simulink model "KUKA_coupled"  (R2021b)
settings: Solver=ode4  StartTime=0.0  StopTime=0.01  FixedStep=0.01  RelTol=1e-3  EnableMultiTasking=on
InitFcn:
  | % ************** Initiate forces
  | % f0=[0;0;0;0;0;0];
  | % f0=[0;0;0;0;0;0;0];
  | %f_0=[0;0;0];
  | %f_m=[0;0];
  | %f_e=[0;0;0;0;0;0];
  | %iota0=eye(6);
  | % ************** Initiate states
  | %q_m=[2;1];
  | %q_dot_m=[0;1];
  | %P=[0;0;0];
  | %V_I0=[0;0;0];
  | % ************** Load main
  | %run(Main.m)
StopFcn:
  | %format long
  | %table(out.qddot.data(:,1)',out.qddot_ref.data(1,:))
values from neighbouring files (symbols this model uses):
  diag_M = diagonalize(M_frak0, M_frak)    [Create_Robot.m]    (also in Main.m; Main__iiwa7.m; diagonalize.m = zeros(6*(n+1),6*(n+1)); test_C_Main.m)
  f_0 = [0;0;0]    [Create_Robot.m]    (also in Main.m; Main__iiwa7.m = [0;0;0;0;0;0]; test_C_Main.m)
  f_e = [0;0;0;0;0;0]    [Create_Robot.m]    (also in Main.m = [0;0;0]; Main__iiwa7.m; test_C_Main.m)
  f_m = [0;0]    [Create_Robot.m]    (also in Main.m; Main__iiwa7.m; test_C_Main.m)
  I0 = eye(3)*416.667    [Create_Robot.m]    (also in Main.m; Main__iiwa7.m = eye(3)*1.66667; test_C_Main.m)
  iota0 = [1 0 0; 0 1 0;zeros(3,3);0 0 1]    [Create_Robot.m]    (also in Main.m = [1 0 0 0 0 0; 0 1 0 0 0 0; 0 0 0 0 0 1]'; Main__iiwa7.m = eye(6,6); test_C_Main.m)
  m0 = 100    [Create_Robot.m]    (also in Main.m; Main__iiwa7.m = 10; test_C_Main.m)
  P = [0;0;0]    [Create_Robot.m]    (also in Main.m = M0*V_I0+M0m*q_dot_m; Main__iiwa7.m = M0*V_I0+M0m*q_dot_m; test_C_Main.m)
  q_dot_m = [0;0]    [Create_Robot.m]    (also in Main.m; Main__iiwa7.m; test_C_Main.m)
  q_m = [0;0]    [Create_Robot.m]    (also in Main.m = [0.2;0.4]; Main__iiwa7.m = [0.2;0.4]; test_C_Main.m = [1;0])
  sc_size = 5    [Main.m]    (also in Main__iiwa7.m = 1)
  X = [0 -x(3) x(2) ; x(3) 0 -x(1) ; -x(2) x(1) 0 ]    [skewsym.m]
  Xi_m_matrix = zeros(6*n,n)    [Create_Robot.m]    (also in Main.m; Main__iiwa7.m; test_C_Main.m)
undefined symbols (not defined in the file or in its folder): rho_0t, V_0t, Xi_m, Y, Z
libraries: sm_lib x87, nesl_utility x51, robotcorelib x2
(part 1 of 3)
settings Model: Creator=Bmmog  LastModifiedBy=Bmmog
settings SimscapeCC: SimscapeLogType=all
settings ExplorerConfigSet: InternalSimMechanicsExplorerSettings="<ExplorerConfiguration><canonicalview>default</canonicalview><AnimationSetting><BasePlaybackSpeed>1.0</BasePlaybackSpeed><PlaybackSpeedFactor>1.0</PlaybackSpeedFactor></AnimationSetting><TilePanel><TileInfo><Tiles Columns=\"1\" Count=\"1\" Rows=\"1\"><Column Weight=\"1\"/><Row Weight=\"1\"/><Tile Height=\"1\" Width=\"1\" X=\"0\" Y=\"0\"/></Tiles></TileInfo><SceneInfo><SceneViewer><BGColor><R>1</R><G>1</G><B>1</B></BGColor><Camera><DoPerspective>off</DoPerspective><Position><X>-2.86799693255843557</X><Y>0.354289043707541051</Y><Z>3.4484382025260043</Z></Position><Center><X>-0.226627357164881998</X><Y>-0.0947422938384068769</Y><Z>1.20474693109606124</Z></Center><Up><X>0.463975295415888944</X><Y>0.796982789726579544</Y><Z>0.386710949060636133</Z></Up><ViewLimDist>1</ViewLimDist><YLim>1.02199972307052578</YLim><XLim>1.06112681813448173</XLim></Camera></SceneViewer></SceneInfo></TilePanel><MechEditorPanel><Cameras/><GfxPanelCameraMap/><VideoCreator><PlaybackSpeedRatio>1.0</PlaybackSpeedRatio><FrameRate>30</FrameRate><VideoFormat>Motion JPEG AVI</VideoFormat><FrameSize>auto</FrameSize></VideoCreator></MechEditorPanel></ExplorerConfiguration>"

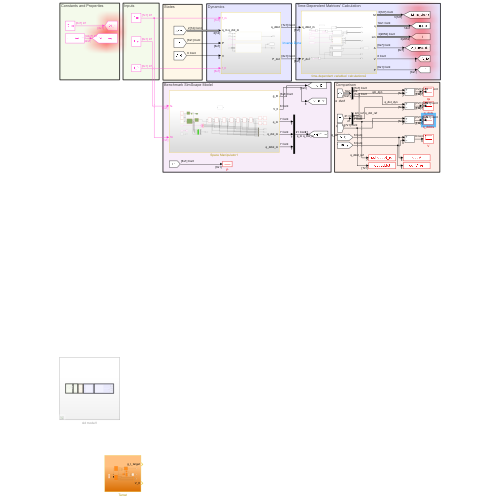
[thumbnail: Simulink's stored preview of the top-level diagram]
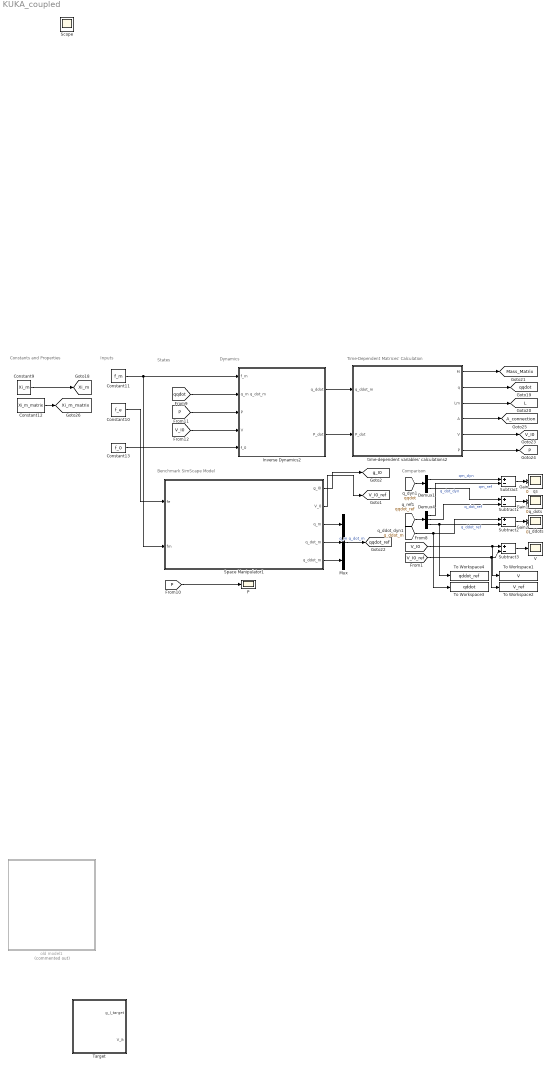
== system KUKA_coupled ==
  note: Benchmark SimScape Model
  note: Time-Dependent Matrices' Calculation
  note: Comparison
  note: States
  note: Constants and Properties
  note: Inputs
  note: Dynamics
  Constant10 : Constant  Value=f_e  VectorParams1D=off
  Constant11 : Constant  Value=f_m  VectorParams1D=off
  Constant12 : Constant  Value=Xi_m_matrix  VectorParams1D=off
  Constant13 : Constant  Value=f_0  VectorParams1D=off
  Constant9 : Constant  Value=Xi_m  VectorParams1D=off
  Demux1 : Demux  Outputs=2
  Demux4 : Demux  Outputs=3
  Gain : Gain  Gain=0
  Gain1 : Gain  Gain=0
  Gain2 : Gain  Gain=0
  Inverse Dynamics2 : Subsystem
  Mux : Mux  Inputs=3
  P : Scope
  Space Manipulator1 : Subsystem
  Subtract{,1..3} (4 alike) : Sum  Inputs=+-
  Target : Subsystem
  To Workspace1 : ToWorkspace  VariableName=V  SaveFormat=Timeseries  SampleTime=-1
  To Workspace2 : ToWorkspace  VariableName=V_ref  SaveFormat=Timeseries  SampleTime=-1
  To Workspace3 : ToWorkspace  VariableName=qddot  SaveFormat=Timeseries  SampleTime=-1
  To Workspace4 : ToWorkspace  VariableName=qddot_ref  SaveFormat=Timeseries  SampleTime=-1
  V : Scope
  old model1 : Subsystem  Commented=on
  q_ddots : Scope
  q_dots : Scope
  qs : Scope
  time-dependent variables' calculations2 : Subsystem
  Scope : Scope
  tag scope: A_connection=global, L=global, Mass_Matrix=global, P=global, V_I0=global, V_I0_ref=global, Xi_m=global, Xi_m_matrix=global, g_I0=global, qqdot=global, qqdot_ref=global
  wires:
  [P] -> P/1
  Constant10/1 -> Space Manipulator1/1(fe)
  Constant12/1 -> [Xi_m_matrix]
  [qqdot] -> Demux1/1
  Inverse Dynamics2/1(q_ddot) -> time-dependent variables' calculations2/1(q_ddot_m)
  Demux1/1 -> Subtract/1  "qm_dyn"
  Demux4/1 -> Subtract/2  "qm_ref"
  [qqdot_ref] -> Demux4/1
  Space Manipulator1/4(q_dot_m) -> Mux/2
  time-dependent variables' calculations2/1(M) -> [Mass_Matrix]
  Constant9/1 -> [Xi_m]
  Constant11/1 -> Space Manipulator1/2(fm), Inverse Dynamics2/1(f_m)
  [q_ddot_m] -> Subtract2/1, To Workspace3/1
  [qqdot] -> Inverse Dynamics2/2(q_m q_dot_m)
  Mux/1 -> [qqdot_ref]  "q_m q_dot_m"
  Demux1/2 -> Subtract1/1  "q_dot_dyn"
  Space Manipulator1/3(q_m) -> Mux/1
  [V_I0] -> Inverse Dynamics2/4(V)
  [V_I0] -> To Workspace1/1, Subtract3/1
  Inverse Dynamics2/2(P_dot) -> time-dependent variables' calculations2/2(P_dot)
  time-dependent variables' calculations2/6(P) -> [P]
  time-dependent variables' calculations2/3(Lm) -> [L]
  [P] -> Inverse Dynamics2/3(P)
  time-dependent variables' calculations2/5(V) -> [V_I0]
  Constant13/1 -> Inverse Dynamics2/5(f_0)
  time-dependent variables' calculations2/4(A) -> [A_connection]
  Demux4/3 -> Subtract2/2, To Workspace4/1  "q_ddot_ref"
  time-dependent variables' calculations2/2(q) -> [qqdot]
  Space Manipulator1/5(q_ddot_m) -> Mux/3
  Demux4/2 -> Subtract1/2  "q_dot_ref"
  Space Manipulator1/2(V_0) -> [V_I0_ref]
  [V_I0_ref] -> To Workspace2/1, Subtract3/2
  Subtract/1 -> Gain/1
  Subtract1/1 -> Gain1/1
  Subtract2/1 -> Gain2/1
  Subtract3/1 -> V/1
  Space Manipulator1/1(g_I0) -> [g_I0]
  Gain/1 -> qs/1
  Gain1/1 -> q_dots/1
  Gain2/1 -> q_ddots/1

== system KUKA_coupled/Inverse Dynamics2 ==
  f_m : Inport
  q_m q_dot_m : Inport  Port=2
  P : Inport  Port=3
  V : Inport  Port=4
  f_0 : Inport  Port=5
  Euler Poincare : Subsystem
  Internal Dynamics : Subsystem
  q_ddot : Outport
  P_dot : Outport  Port=2
  tag scope: q_ddot_m=global
  wires:
  f_m/1 -> Internal Dynamics/1(f_m)
  q_m q_dot_m/1 -> Internal Dynamics/2(q_m q_dot_m)
  Internal Dynamics/1(q_ddot) -> [q_ddot_m], q_ddot/1  "q_ddot"
  Euler Poincare/1(P_dot) -> P_dot/1  "P_dot"
  f_0/1 -> Euler Poincare/3(f_0)
  P/1 -> Internal Dynamics/3(P), Euler Poincare/1(P)
  V/1 -> Euler Poincare/2(V)

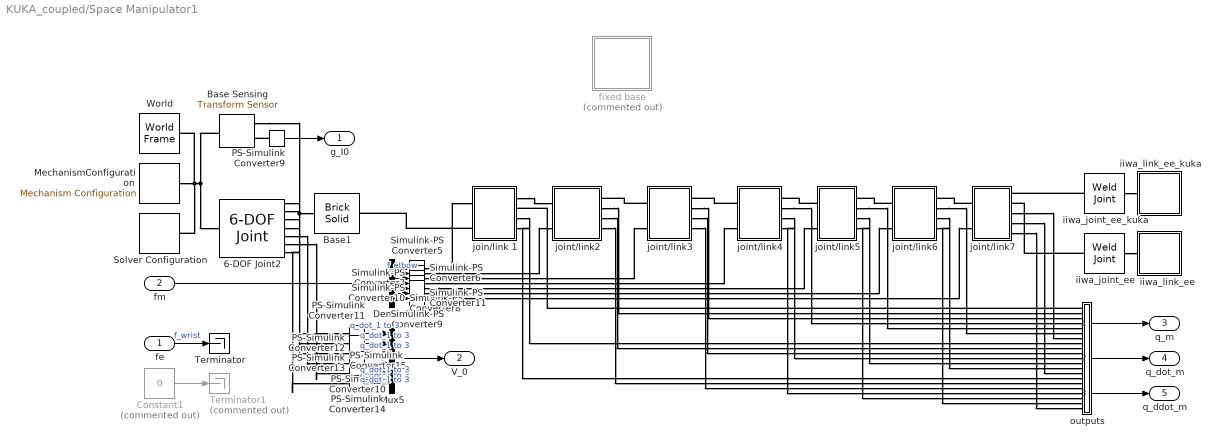
== system KUKA_coupled/Space Manipulator1 ==
  fe : Inport
  fm : Inport  Port=2
  6-DOF Joint2 : sm_lib/Joints/6-DOF Joint  JointMode=Normal  SenseConstraintForce=off  SenseConstraintForceX=off  SenseConstraintForceY=off  SenseConstraintForceZ=off  SenseConstraintTorque=off  SenseConstraintTorqueX=off  SenseConstraintTorqueY=off  SenseConstraintTorqueZ=off  SenseTotalForce=off  SenseTotalForceX=off  SenseTotalForceY=off  SenseTotalForceZ=off  SenseTotalTorque=off  SenseTotalTorqueX=off  SenseTotalTorqueY=off  SenseTotalTorqueZ=off  CompositeWrenchDir=FollowerOnBase  CompositeWrenchFrame=BaseFrame  PxEquilibriumPosition=0  PxEquilibriumPositionUnits=m  PxSpringStiffness=0  PxSpringStiffnessUnits=N/m  PxDampingCoefficient=0  PxDampingCoefficientUnits=N/(m/s)  PxTorqueActuationMode=NoTorque  PxMotionActuationMode=ComputedMotion  PxSensePosition=off  PxSenseVelocity=on  PxSenseAcceleration=off  PxSenseTorqueForce=off  PxSenseLowerLimitTorqueForce=off  PxSenseUpperLimitTorqueForce=off  PxLowerLimitSpecify=off  PxLowerLimitBound=-1  PxLowerLimitBoundUnits=m  PxLowerLimitStiffness=1e6  PxLowerLimitStiffnessUnits=N/m  PxLowerLimitDamping=1e3  PxLowerLimitDampingUnits=N/(m/s)  PxLowerLimitTransitionRegionWidth=1e-4  PxLowerLimitTransitionRegionWidthUnits=m  PxUpperLimitSpecify=off  PxUpperLimitBound=1  PxUpperLimitBoundUnits=m  PxUpperLimitStiffness=1e6  PxUpperLimitStiffnessUnits=N/m  PxUpperLimitDamping=1e3  PxUpperLimitDampingUnits=N/(m/s)  PxUpperLimitTransitionRegionWidth=1e-4  PxUpperLimitTransitionRegionWidthUnits=m  PxPositionTargetSpecify=on  PxPositionTargetPriority=High  PxPositionTargetValue=0  PxPositionTargetValueUnits=m  PxVelocityTargetSpecify=off  PxVelocityTargetPriority=High  PxVelocityTargetValue=0  PxVelocityTargetValueUnits=m/s  PyEquilibriumPosition=0  PyEquilibriumPositionUnits=m  PySpringStiffness=0  PySpringStiffnessUnits=N/m  PyDampingCoefficient=0  PyDampingCoefficientUnits=N/(m/s)  PyTorqueActuationMode=NoTorque  PyMotionActuationMode=ComputedMotion  PySensePosition=off  PySenseVelocity=on  PySenseAcceleration=off  PySenseTorqueForce=off  PySenseLowerLimitTorqueForce=off  PySenseUpperLimitTorqueForce=off  PyLowerLimitSpecify=off  PyLowerLimitBound=-1  PyLowerLimitBoundUnits=m  PyLowerLimitStiffness=1e6  PyLowerLimitStiffnessUnits=N/m  PyLowerLimitDamping=1e3  PyLowerLimitDampingUnits=N/(m/s)  PyLowerLimitTransitionRegionWidth=1e-4  PyLowerLimitTransitionRegionWidthUnits=m  PyUpperLimitSpecify=off  PyUpperLimitBound=1  PyUpperLimitBoundUnits=m  PyUpperLimitStiffness=1e6  PyUpperLimitStiffnessUnits=N/m  PyUpperLimitDamping=1e3  PyUpperLimitDampingUnits=N/(m/s)  PyUpperLimitTransitionRegionWidth=1e-4  PyUpperLimitTransitionRegionWidthUnits=m  PyPositionTargetSpecify=on  PyPositionTargetPriority=High  PyPositionTargetValue=0  PyPositionTargetValueUnits=m  PyVelocityTargetSpecify=off  PyVelocityTargetPriority=High  PyVelocityTargetValue=0  PyVelocityTargetValueUnits=m/s  PzEquilibriumPosition=0  PzEquilibriumPositionUnits=m  PzSpringStiffness=0  PzSpringStiffnessUnits=N/m  PzDampingCoefficient=0  PzDampingCoefficientUnits=N/(m/s)  PzTorqueActuationMode=NoTorque  PzMotionActuationMode=ComputedMotion  PzSensePosition=off  PzSenseVelocity=on  PzSenseAcceleration=off  PzSenseTorqueForce=off  PzSenseLowerLimitTorqueForce=off  PzSenseUpperLimitTorqueForce=off  PzLowerLimitSpecify=off  PzLowerLimitBound=-1  PzLowerLimitBoundUnits=m  PzLowerLimitStiffness=1e6  PzLowerLimitStiffnessUnits=N/m  PzLowerLimitDamping=1e3  PzLowerLimitDampingUnits=N/(m/s)  PzLowerLimitTransitionRegionWidth=1e-4  PzLowerLimitTransitionRegionWidthUnits=m  PzUpperLimitSpecify=off  PzUpperLimitBound=1  PzUpperLimitBoundUnits=m  PzUpperLimitStiffness=1e6  PzUpperLimitStiffnessUnits=N/m  PzUpperLimitDamping=1e3  PzUpperLimitDampingUnits=N/(m/s)  PzUpperLimitTransitionRegionWidth=1e-4  PzUpperLimitTransitionRegionWidthUnits=m  PzPositionTargetSpecify=on  PzPositionTargetPriority=High  PzPositionTargetValue=0  PzPositionTargetValueUnits=m  PzVelocityTargetSpecify=off  PzVelocityTargetPriority=High  PzVelocityTargetValue=0  PzVelocityTargetValueUnits=m/s  SphDefPosRotationMethod=None  SphDefPosRotationAngleUnits=deg  SphDefPosRotationStandardAxis=+Z  SphDefPosRotationAngle=0.0  SphDefPosRotationArbitraryAxis=[0 0 1]  SphDefPosFollAlignAxisA=+X  SphDefPosBaseAlignAxisA=+Y  SphDefPosFollAlignAxisB=+Y  SphDefPosBaseAlignAxisB=+Z  SphDefPosRotationSequenceAxes=FollowerAxes  SphDefPosRotationSequence=XYX  SphDefPosRotationSequenceAngles=[0 0 0]  SphDefPosRotationSequenceAnglesUnits=deg  SphDefPosRotationMatrix=[1 0 0; 0 1 0; 0 0 1]  SphEqPosRotationMethod=None  SphEqPosRotationAngleUnits=deg  SphEqPosRotationStandardAxis=+Z  SphEqPosRotationAngle=0.0  SphEqPosRotationArbitraryAxis=[0 0 1]  SphEqPosFollAlignAxisA=+X  SphEqPosBaseAlignAxisA=+Y  SphEqPosFollAlignAxisB=+Y  SphEqPosBaseAlignAxisB=+Z  SphEqPosRotationSequenceAxes=FollowerAxes  SphEqPosRotationSequence=XYX  SphEqPosRotationSequenceAngles=[0 0 0]  SphEqPosRotationSequenceAnglesUnits=deg  SphEqPosRotationMatrix=[1 0 0; 0 1 0; 0 0 1]  SphSpringStiffness=0  SphSpringStiffnessUnits=N*m/deg  SphDampingCoefficient=0  SphDampingCoefficientUnits=N*m/(deg/s)  SphActuateTorqueX=off  SphActuateTorqueY=off  SphActuateTorqueZ=off  SphActuateTorque=off  SphTorqueActuationMode=NoTorque  SphMotionActuationMode=ComputedMotion  SphActuationFrame=BaseFrame  SphSensePosition=off  SphSenseVelocityX=on  SphSenseVelocityY=on  SphSenseVelocityZ=on  SphSenseVelocity=off  SphSenseAccelerationX=off  SphSenseAccelerationY=off  SphSenseAccelerationZ=off  SphSenseAcceleration=off  SphSenseTorqueX=off  SphSenseTorqueY=off  SphSenseTorqueZ=off  SphSenseTorqueForce=off  SphSenseLowerLimitTorqueMag=off  SphSenseUpperLimitTorqueMag=off  SphSensingFrame=BaseFrame  SphLowerLimitSpecify=off  SphLowerLimitBound=15  SphLowerLimitBoundUnits=deg  SphLowerLimitStiffness=1e4  SphLowerLimitStiffnessUnits=N*m/deg  SphLowerLimitDamping=10  SphLowerLimitDampingUnits=N*m/(deg/s)  SphLowerLimitTransitionRegionWidth=0.1  SphLowerLimitTransitionRegionWidthUnits=deg  SphUpperLimitSpecify=off  SphUpperLimitBound=45  SphUpperLimitBoundUnits=deg  SphUpperLimitStiffness=1e4  SphUpperLimitStiffnessUnits=N*m/deg  SphUpperLimitDamping=10  SphUpperLimitDampingUnits=N*m/(deg/s)  SphUpperLimitTransitionRegionWidth=0.1  SphUpperLimitTransitionRegionWidthUnits=deg  SphPositionTargetRotationMethod=RotationSequence  SphPositionTargetRotationAngleUnits=deg  SphPositionTargetRotationStandardAxis=+Z  SphPositionTargetRotationAngle=0.0  SphPositionTargetRotationArbitraryAxis=[0 0 1]  SphPositionTargetFollAlignAxisA=+X  SphPositionTargetBaseAlignAxisA=+Y  SphPositionTargetFollAlignAxisB=+Y  SphPositionTargetBaseAlignAxisB=+Z  SphPositionTargetRotationSequenceAxes=FollowerAxes  SphPositionTargetRotationSequence=ZYX  SphPositionTargetRotationSequenceAngles=[0 0 0]  SphPositionTargetRotationSequenceAnglesUnits=deg  SphPositionTargetRotationMatrix=[1 0 0; 0 1 0; 0 0 1]  SphPositionTargetSpecify=off  SphPositionTargetPriority=High  SphVelocityTargetValue=[0 0.5 0.5]  SphVelocityTargetValueUnits=rad/s  SphVelocityTargetSpecify=off  SphVelocityTargetPriority=High  SphVelocityTargetInFollowerFrame=on
  Base Sensing : sm_lib/Frames and Transforms/Transform Sensor  MeasurementFrame=Base  SenseAngle=off  SenseAxis=off  SenseAngle1=off  SenseAngle2=off  SenseAngle3=off  SenseQ=off  SenseR=on  SenseOmegaX=off  SenseOmegaY=off  SenseOmegaZ=off  SenseOmega1=off  SenseOmega2=off  SenseOmega3=off  SenseQDot=off  SenseRDot=off  SenseAlphaX=off  SenseAlphaY=off  SenseAlphaZ=off  SenseAlpha1=off  SenseAlpha2=off  SenseAlpha3=off  SenseQDDot=off  SenseRDDot=off  SenseX=off  SenseY=off  SenseZ=off  SenseRad=off  SenseAzim=off  SenseDist=off  SenseInc=off  SenseXDot=off  SenseYDot=off  SenseZDot=off  SenseRadDot=off  SenseAzimDot=off  SenseDistDot=off  SenseIncDot=off  SenseXDDot=off  SenseYDDot=off  SenseZDDot=off  SenseRadDDot=off  SenseAzimDDot=off  SenseDistDDot=off  SenseIncDDot=off
  Base1 : sm_lib/Body Elements/Brick Solid  GraphicAmbientColor=[0.15 0.15 0.15 1.0]  BasedOnType=Mass  BrickDimensions=[sc_size,sc_size,sc_size]  BrickDimensionUnits=m  CenterOfMass=[0 0 0]  CenterOfMassUnits=m  GraphicDiffuseColor=[0.5 0.5 0.5]  Density=1000  DensityUnits=kg/m^3  DoExposeReferenceFrame=on  GraphicEmissiveColor=[0.0 0.0 0.0 1.0]  ExportEntireGeometry=off  SerializedFrames=<Frames><Frame><Id>Frame1</Id><Value><Name>F1</Name><Origin><Source>GeometricFeature</Source><FeatureName>+z surface</FeatureName></Origin><PrimaryAxis><DefinedDirection>+X</DefinedDirection><Source>ReferenceFrame</Source><SourceDirection>+X</SourceDirection><FeatureName></FeatureName></PrimaryAxis><SecondaryAxis><DefinedDirection>+Z</DefinedDirection><Source>ReferenceFrame</Source><SourceDirection>+Z</SourceDirection><FeatureName></FeatureName></SecondaryAxis></Value></Frame></Frames>  MarkerShape=Sphere  MarkerSize=10  GraphicType=FromGeometry  InertiaType=CalculateFromGeometry  Mass=m0  MassUnits=kg  MomentsOfInertia=[I0(1,1) I0(2,2) I0(3,3)]  MomentsOfInertiaUnits=kg*m^2  GraphicOpacity=1.0  ProductsOfInertia=[0 0 0]  ProductsOfInertiaUnits=kg*m^2  GraphicShininess=75  GraphicSpecularColor=[0.5 0.5 0.5 1.0]  GraphicVisPropType=SimpleVisualProperties
  Constant1 : Constant  Commented=on  Value=0
  Demux2 : Demux  Outputs=7
  MechanismConfiguration : sm_lib/Utilities/Mechanism Configuration  UniformGravity=Constant  GravityVector=[0 0 0]  GravityUnits=m/s^2  LinearizationDelta=0.001  JointModeTransitionNonlinearIterations=2
  Mux5 : Mux  Inputs=6
  PS-Simulink Converter{9..15} (7 alike) : nesl_utility/PS-Simulink Converter  PhysicalDomain=network_engine_domain  SubClassName=ps_output  LeftPortType=input  RightPortType=output  PseudoPeriodic=off  Frequencies=[]  Unit=inherit  AffineConversion=off
      settings: SourceProductBaseCode=PW,SS
  Simulink-PS Converter{5..11} (7 alike) : nesl_utility/Simulink-PS Converter  PhysicalDomain=network_engine_domain  SubClassName=ps_input  LeftPortType=input  RightPortType=output  PseudoPeriodic=off  Frequencies=[]  NoiseDistribution=none  NoiseParameters=[]  Unit=1  AffineConversion=off  FilteringAndDerivatives=provide  SimscapeFilterOrder=1  InputFilterTimeConstant=0.001  UdotUserProvided=0
      settings: SourceProductBaseCode=PW,SS
  Solver Configuration : nesl_utility/Solver Configuration  PhysicalDomain=network_engine_domain  SubClassName=solver  LeftPortType=input  RightPortType=generic  Tones=[]  Harmonics=[]  SimulateNoise=off  Profile=off  UseLocalSampling=off  EnableSwitchedLinearOptims=on  FrequencyDomain=off  UseCCode=off  RelTol=0.001  AbsTol=0.001  MinStep=1e-09  ToWorkspace=off  RevertToSquareIcSolve=off  NumHomotopyIterations=100  PhasorMode=off  PhasorModeNumHarmonics=1  DoDC=off  ResidualTolerance=1e-09  UseLocalSolver=off  LocalSolverChoice=NE_BACKWARD_EULER_ADVANCER  LocalSolverSampleTime=0.001  DoFixedCost=off  MaxNonlinIter=3  MaxModeIter=2  ComputeImpulses=off  ImpulseIterations=2  LinearAlgebra=auto  EquationFormulation=NE_TIME_EF  DelaysMemoryBudget=1024  AutomaticFiltering=on  FilteringTimeConstant=0.001  PartitionStorageMethod=AS_NEEDED  PartitionMemoryBudget=1024  PartitionMethod=ROBUST
      settings: SourceProductBaseCode=PW,SS
  Terminator : Terminator
  Terminator1 : Terminator  Commented=on
  World : sm_lib/Frames and Transforms/World Frame
  fixed base : Subsystem  Commented=on
  iiwa_joint_ee : sm_lib/Joints/Weld Joint  JointMode=Normal  SenseConstraintForce=off  SenseConstraintForceX=off  SenseConstraintForceY=off  SenseConstraintForceZ=off  SenseConstraintTorque=off  SenseConstraintTorqueX=off  SenseConstraintTorqueY=off  SenseConstraintTorqueZ=off  SenseTotalForce=off  SenseTotalForceX=off  SenseTotalForceY=off  SenseTotalForceZ=off  SenseTotalTorque=off  SenseTotalTorqueX=off  SenseTotalTorqueY=off  SenseTotalTorqueZ=off  CompositeWrenchDir=FollowerOnBase  CompositeWrenchFrame=BaseFrame
  iiwa_joint_ee_kuka : sm_lib/Joints/Weld Joint  JointMode=Normal  SenseConstraintForce=off  SenseConstraintForceX=off  SenseConstraintForceY=off  SenseConstraintForceZ=off  SenseConstraintTorque=off  SenseConstraintTorqueX=off  SenseConstraintTorqueY=off  SenseConstraintTorqueZ=off  SenseTotalForce=off  SenseTotalForceX=off  SenseTotalForceY=off  SenseTotalForceZ=off  SenseTotalTorque=off  SenseTotalTorqueX=off  SenseTotalTorqueY=off  SenseTotalTorqueZ=off  CompositeWrenchDir=FollowerOnBase  CompositeWrenchFrame=BaseFrame
  iiwa_link_ee : Subsystem
  iiwa_link_ee_kuka : Subsystem
  join/link 1 : Subsystem
  joint/link2 : Subsystem
  joint/link3 : Subsystem
  joint/link4 : Subsystem
  joint/link5 : Subsystem
  joint/link6 : Subsystem
  joint/link7 : Subsystem
  outputs : Subsystem
  g_I0 : Outport
  V_0 : Outport  Port=2
  q_m : Outport  Port=3
  q_dot_m : Outport  Port=4
  q_ddot_m : Outport  Port=5
  wires:
  fe/1 -> Terminator/1  "f_wrist"
  Constant1/1 -> Terminator1/1
  PS-Simulink Converter12/1 -> Mux5/2  "q_dot_1 to 3"
  PS-Simulink Converter15/1 -> Mux5/6  "q_dot_1 to 3"
  Mux5/1 -> V_0/1
  PS-Simulink Converter13/1 -> Mux5/4  "q_dot_1 to 3"
  PS-Simulink Converter9/1 -> g_I0/1
  PS-Simulink Converter11/1 -> Mux5/1  "q_dot_1 to 3"
  PS-Simulink Converter14/1 -> Mux5/5  "q_dot_1 to 3"
  PS-Simulink Converter10/1 -> Mux5/3  "q_dot_1 to 3"
  fm/1 -> Demux2/1
  Demux2/3 -> Simulink-PS Converter7/1
  Demux2/1 -> Simulink-PS Converter5/1
  Demux2/6 -> Simulink-PS Converter10/1
  Demux2/5 -> Simulink-PS Converter9/1
  Demux2/2 -> Simulink-PS Converter6/1  "f_elbow"
  Demux2/4 -> Simulink-PS Converter8/1
  outputs/2(q_dot_m) -> q_dot_m/1
  outputs/1(q_m) -> q_m/1
  outputs/3(q_ddot_m) -> q_ddot_m/1
  Demux2/7 -> Simulink-PS Converter11/1
  connections:
  Base1/RConn1 -- 6-DOF Joint2/RConn1 -- Base Sensing/RConn1
  MechanismConfiguration/RConn1 -- 6-DOF Joint2/LConn1 -- Base Sensing/LConn1 -- Solver Configuration/RConn1 -- World/RConn1
  6-DOF Joint2/RConn4 -- PS-Simulink Converter10/LConn1
  6-DOF Joint2/RConn6 -- PS-Simulink Converter14/LConn1
  6-DOF Joint2/RConn7 -- PS-Simulink Converter15/LConn1
  PS-Simulink Converter9/LConn1 -- Base Sensing/RConn2
  6-DOF Joint2/RConn2 -- PS-Simulink Converter11/LConn1
  6-DOF Joint2/RConn3 -- PS-Simulink Converter12/LConn1
  6-DOF Joint2/RConn5 -- PS-Simulink Converter13/LConn1
  joint/link6/LConn1 -- joint/link5/RConn1
  iiwa_joint_ee/LConn1 -- joint/link7/RConn2
  joint/link3/RConn4 -- outputs/LConn17
  Simulink-PS Converter5/RConn1 -- join/link 1/LConn1
  Simulink-PS Converter10/RConn1 -- joint/link6/LConn2
  join/link 1/RConn4 -- outputs/LConn15
  joint/link3/RConn2 -- outputs/LConn3
  joint/link7/RConn5 -- outputs/LConn21
  joint/link7/RConn3 -- outputs/LConn7
  joint/link6/RConn4 -- outputs/LConn20
  joint/link4/RConn4 -- outputs/LConn18
  joint/link3/LConn1 -- joint/link2/RConn1
  Simulink-PS Converter8/RConn1 -- joint/link4/LConn2
  Simulink-PS Converter6/RConn1 -- joint/link2/LConn2
  joint/link2/RConn4 -- outputs/LConn16
  joint/link2/RConn2 -- outputs/LConn2
  joint/link4/RConn3 -- outputs/LConn11
  joint/link6/RConn3 -- outputs/LConn13
  joint/link7/LConn1 -- joint/link6/RConn1
  iiwa_joint_ee_kuka/RConn1 -- iiwa_link_ee_kuka/LConn1
  joint/link5/RConn3 -- outputs/LConn12
  joint/link6/RConn2 -- outputs/LConn6
  joint/link5/RConn4 -- outputs/LConn19
  joint/link7/RConn4 -- outputs/LConn14
  iiwa_joint_ee/RConn1 -- iiwa_link_ee/LConn1
  Simulink-PS Converter9/RConn1 -- joint/link5/LConn2
  joint/link3/RConn3 -- outputs/LConn10
  join/link 1/RConn1 -- joint/link2/LConn1
  join/link 1/LConn2 -- Base1/LConn1
  iiwa_joint_ee_kuka/LConn1 -- joint/link7/RConn1
  joint/link5/RConn2 -- outputs/LConn5
  joint/link4/LConn1 -- joint/link3/RConn1
  joint/link2/RConn3 -- outputs/LConn9
  joint/link4/RConn2 -- outputs/LConn4
  Simulink-PS Converter11/RConn1 -- joint/link7/LConn2
  joint/link5/LConn1 -- joint/link4/RConn1
  outputs/LConn1 -- join/link 1/RConn2
  join/link 1/RConn3 -- outputs/LConn8
  Simulink-PS Converter7/RConn1 -- joint/link3/LConn2

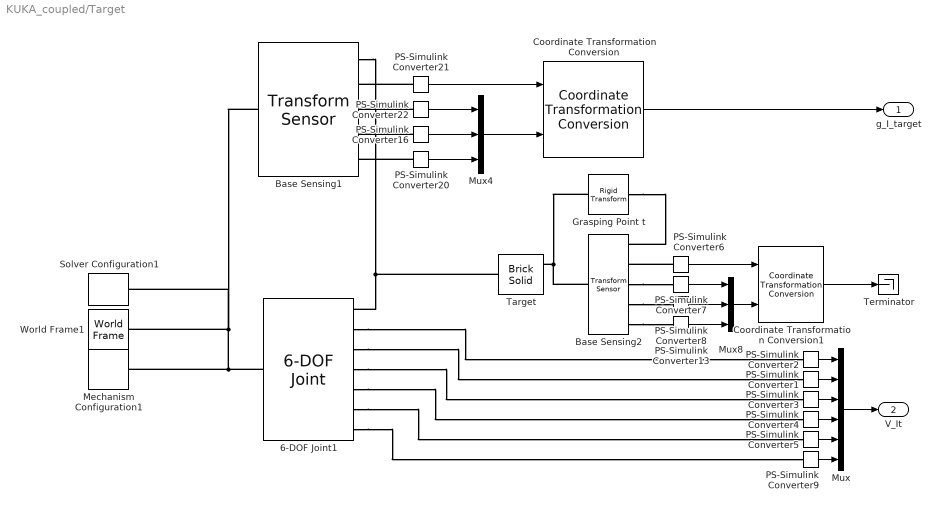
== system KUKA_coupled/Target ==
  6-DOF Joint1 : sm_lib/Joints/6-DOF Joint  JointMode=Normal  SenseConstraintForce=off  SenseConstraintForceX=off  SenseConstraintForceY=off  SenseConstraintForceZ=off  SenseConstraintTorque=off  SenseConstraintTorqueX=off  SenseConstraintTorqueY=off  SenseConstraintTorqueZ=off  SenseTotalForce=off  SenseTotalForceX=off  SenseTotalForceY=off  SenseTotalForceZ=off  SenseTotalTorque=off  SenseTotalTorqueX=off  SenseTotalTorqueY=off  SenseTotalTorqueZ=off  CompositeWrenchDir=FollowerOnBase  CompositeWrenchFrame=BaseFrame  PxEquilibriumPosition=0  PxEquilibriumPositionUnits=m  PxSpringStiffness=0  PxSpringStiffnessUnits=N/m  PxDampingCoefficient=0  PxDampingCoefficientUnits=N/(m/s)  PxTorqueActuationMode=NoTorque  PxMotionActuationMode=ComputedMotion  PxSensePosition=off  PxSenseVelocity=on  PxSenseAcceleration=off  PxSenseTorqueForce=off  PxSenseLowerLimitTorqueForce=off  PxSenseUpperLimitTorqueForce=off  PxLowerLimitSpecify=off  PxLowerLimitBound=-1  PxLowerLimitBoundUnits=m  PxLowerLimitStiffness=1e6  PxLowerLimitStiffnessUnits=N/m  PxLowerLimitDamping=1e3  PxLowerLimitDampingUnits=N/(m/s)  PxLowerLimitTransitionRegionWidth=1e-4  PxLowerLimitTransitionRegionWidthUnits=m  PxUpperLimitSpecify=off  PxUpperLimitBound=1  PxUpperLimitBoundUnits=m  PxUpperLimitStiffness=1e6  PxUpperLimitStiffnessUnits=N/m  PxUpperLimitDamping=1e3  PxUpperLimitDampingUnits=N/(m/s)  PxUpperLimitTransitionRegionWidth=1e-4  PxUpperLimitTransitionRegionWidthUnits=m  PxPositionTargetSpecify=on  PxPositionTargetPriority=High  PxPositionTargetValue=rho_0t(1)  PxPositionTargetValueUnits=m  PxVelocityTargetSpecify=on  PxVelocityTargetPriority=High  PxVelocityTargetValue=V_0t(1)  PxVelocityTargetValueUnits=m/s  PyEquilibriumPosition=0  PyEquilibriumPositionUnits=m  PySpringStiffness=0  PySpringStiffnessUnits=N/m  PyDampingCoefficient=0  PyDampingCoefficientUnits=N/(m/s)  PyTorqueActuationMode=NoTorque  PyMotionActuationMode=ComputedMotion  PySensePosition=off  PySenseVelocity=on  PySenseAcceleration=off  PySenseTorqueForce=off  PySenseLowerLimitTorqueForce=off  PySenseUpperLimitTorqueForce=off  PyLowerLimitSpecify=off  PyLowerLimitBound=-1  PyLowerLimitBoundUnits=m  PyLowerLimitStiffness=1e6  PyLowerLimitStiffnessUnits=N/m  PyLowerLimitDamping=1e3  PyLowerLimitDampingUnits=N/(m/s)  PyLowerLimitTransitionRegionWidth=1e-4  PyLowerLimitTransitionRegionWidthUnits=m  PyUpperLimitSpecify=off  PyUpperLimitBound=1  PyUpperLimitBoundUnits=m  PyUpperLimitStiffness=1e6  PyUpperLimitStiffnessUnits=N/m  PyUpperLimitDamping=1e3  PyUpperLimitDampingUnits=N/(m/s)  PyUpperLimitTransitionRegionWidth=1e-4  PyUpperLimitTransitionRegionWidthUnits=m  PyPositionTargetSpecify=on  PyPositionTargetPriority=High  PyPositionTargetValue=rho_0t(2)  PyPositionTargetValueUnits=m  PyVelocityTargetSpecify=on  PyVelocityTargetPriority=High  PyVelocityTargetValue=V_0t(2)  PyVelocityTargetValueUnits=m/s  PzEquilibriumPosition=0  PzEquilibriumPositionUnits=m  PzSpringStiffness=0  PzSpringStiffnessUnits=N/m  PzDampingCoefficient=0  PzDampingCoefficientUnits=N/(m/s)  PzTorqueActuationMode=NoTorque  PzMotionActuationMode=ComputedMotion  PzSensePosition=off  PzSenseVelocity=on  PzSenseAcceleration=off  PzSenseTorqueForce=off  PzSenseLowerLimitTorqueForce=off  PzSenseUpperLimitTorqueForce=off  PzLowerLimitSpecify=off  PzLowerLimitBound=-1  PzLowerLimitBoundUnits=m  PzLowerLimitStiffness=1e6  PzLowerLimitStiffnessUnits=N/m  PzLowerLimitDamping=1e3  PzLowerLimitDampingUnits=N/(m/s)  PzLowerLimitTransitionRegionWidth=1e-4  PzLowerLimitTransitionRegionWidthUnits=m  PzUpperLimitSpecify=off  PzUpperLimitBound=1  PzUpperLimitBoundUnits=m  PzUpperLimitStiffness=1e6  PzUpperLimitStiffnessUnits=N/m  PzUpperLimitDamping=1e3  PzUpperLimitDampingUnits=N/(m/s)  PzUpperLimitTransitionRegionWidth=1e-4  PzUpperLimitTransitionRegionWidthUnits=m  PzPositionTargetSpecify=on  PzPositionTargetPriority=High  PzPositionTargetValue=rho_0t(3)  PzPositionTargetValueUnits=m  PzVelocityTargetSpecify=on  PzVelocityTargetPriority=High  PzVelocityTargetValue=V_0t(3)  PzVelocityTargetValueUnits=m/s  SphDefPosRotationMethod=None  SphDefPosRotationAngleUnits=deg  SphDefPosRotationStandardAxis=+Z  SphDefPosRotationAngle=0.0  SphDefPosRotationArbitraryAxis=[0 0 1]  SphDefPosFollAlignAxisA=+X  SphDefPosBaseAlignAxisA=+Y  SphDefPosFollAlignAxisB=+Y  SphDefPosBaseAlignAxisB=+Z  SphDefPosRotationSequenceAxes=FollowerAxes  SphDefPosRotationSequence=XYX  SphDefPosRotationSequenceAngles=[0 0 0]  SphDefPosRotationSequenceAnglesUnits=deg  SphDefPosRotationMatrix=[1 0 0; 0 1 0; 0 0 1]  SphEqPosRotationMethod=None  SphEqPosRotationAngleUnits=deg  SphEqPosRotationStandardAxis=+Z  SphEqPosRotationAngle=0.0  SphEqPosRotationArbitraryAxis=[0 0 1]  SphEqPosFollAlignAxisA=+X  SphEqPosBaseAlignAxisA=+Y  SphEqPosFollAlignAxisB=+Y  SphEqPosBaseAlignAxisB=+Z  SphEqPosRotationSequenceAxes=FollowerAxes  SphEqPosRotationSequence=XYX  SphEqPosRotationSequenceAngles=[0 0 0]  SphEqPosRotationSequenceAnglesUnits=deg  SphEqPosRotationMatrix=[1 0 0; 0 1 0; 0 0 1]  SphSpringStiffness=0  SphSpringStiffnessUnits=N*m/deg  SphDampingCoefficient=0  SphDampingCoefficientUnits=N*m/(deg/s)  SphActuateTorqueX=off  SphActuateTorqueY=off  SphActuateTorqueZ=off  SphActuateTorque=off  SphTorqueActuationMode=NoTorque  SphMotionActuationMode=ComputedMotion  SphActuationFrame=BaseFrame  SphSensePosition=off  SphSenseVelocityX=on  SphSenseVelocityY=on  SphSenseVelocityZ=on  SphSenseVelocity=off  SphSenseAccelerationX=off  SphSenseAccelerationY=off  SphSenseAccelerationZ=off  SphSenseAcceleration=off  SphSenseTorqueX=off  SphSenseTorqueY=off  SphSenseTorqueZ=off  SphSenseTorqueForce=off  SphSenseLowerLimitTorqueMag=off  SphSenseUpperLimitTorqueMag=off  SphSensingFrame=BaseFrame  SphLowerLimitSpecify=off  SphLowerLimitBound=15  SphLowerLimitBoundUnits=deg  SphLowerLimitStiffness=1e4  SphLowerLimitStiffnessUnits=N*m/deg  SphLowerLimitDamping=10  SphLowerLimitDampingUnits=N*m/(deg/s)  SphLowerLimitTransitionRegionWidth=0.1  SphLowerLimitTransitionRegionWidthUnits=deg  SphUpperLimitSpecify=off  SphUpperLimitBound=45  SphUpperLimitBoundUnits=deg  SphUpperLimitStiffness=1e4  SphUpperLimitStiffnessUnits=N*m/deg  SphUpperLimitDamping=10  SphUpperLimitDampingUnits=N*m/(deg/s)  SphUpperLimitTransitionRegionWidth=0.1  SphUpperLimitTransitionRegionWidthUnits=deg  SphPositionTargetRotationMethod=RotationSequence  SphPositionTargetRotationAngleUnits=deg  SphPositionTargetRotationStandardAxis=+Z  SphPositionTargetRotationAngle=0.0  SphPositionTargetRotationArbitraryAxis=[0 0 1]  SphPositionTargetFollAlignAxisA=+X  SphPositionTargetBaseAlignAxisA=+Y  SphPositionTargetFollAlignAxisB=+Y  SphPositionTargetBaseAlignAxisB=+Z  SphPositionTargetRotationSequenceAxes=FollowerAxes  SphPositionTargetRotationSequence=XYZ  SphPositionTargetRotationSequenceAngles=[45 45 45]  SphPositionTargetRotationSequenceAnglesUnits=deg  SphPositionTargetRotationMatrix=[1 0 0; 0 1 0; 0 0 1]  SphPositionTargetSpecify=on  SphPositionTargetPriority=High  SphVelocityTargetValue=w_t  SphVelocityTargetValueUnits=rad/s  SphVelocityTargetSpecify=on  SphVelocityTargetPriority=High  SphVelocityTargetInFollowerFrame=off
  Base Sensing1 : sm_lib/Frames and Transforms/Transform Sensor  MeasurementFrame=Base  SenseAngle=off  SenseAxis=off  SenseAngle1=off  SenseAngle2=off  SenseAngle3=off  SenseQ=off  SenseR=on  SenseOmegaX=off  SenseOmegaY=off  SenseOmegaZ=off  SenseOmega1=off  SenseOmega2=off  SenseOmega3=off  SenseQDot=off  SenseRDot=off  SenseAlphaX=off  SenseAlphaY=off  SenseAlphaZ=off  SenseAlpha1=off  SenseAlpha2=off  SenseAlpha3=off  SenseQDDot=off  SenseRDDot=off  SenseX=on  SenseY=on  SenseZ=on  SenseRad=off  SenseAzim=off  SenseDist=off  SenseInc=off  SenseXDot=off  SenseYDot=off  SenseZDot=off  SenseRadDot=off  SenseAzimDot=off  SenseDistDot=off  SenseIncDot=off  SenseXDDot=off  SenseYDDot=off  SenseZDDot=off  SenseRadDDot=off  SenseAzimDDot=off  SenseDistDDot=off  SenseIncDDot=off
  Base Sensing2 : sm_lib/Frames and Transforms/Transform Sensor  MeasurementFrame=Base  SenseAngle=off  SenseAxis=off  SenseAngle1=off  SenseAngle2=off  SenseAngle3=off  SenseQ=off  SenseR=on  SenseOmegaX=off  SenseOmegaY=off  SenseOmegaZ=off  SenseOmega1=off  SenseOmega2=off  SenseOmega3=off  SenseQDot=off  SenseRDot=off  SenseAlphaX=off  SenseAlphaY=off  SenseAlphaZ=off  SenseAlpha1=off  SenseAlpha2=off  SenseAlpha3=off  SenseQDDot=off  SenseRDDot=off  SenseX=on  SenseY=on  SenseZ=on  SenseRad=off  SenseAzim=off  SenseDist=off  SenseInc=off  SenseXDot=off  SenseYDot=off  SenseZDot=off  SenseRadDot=off  SenseAzimDot=off  SenseDistDot=off  SenseIncDot=off  SenseXDDot=off  SenseYDDot=off  SenseZDDot=off  SenseRadDDot=off  SenseAzimDDot=off  SenseDistDDot=off  SenseIncDDot=off
  Coordinate Transformation Conversion : robotcorelib/Coordinate Transformation Conversion  InputRepresentation=Rotation Matrix  InputEulerSequence=ZYX  ShowTrVecInputPort=on  OutputRepresentation=Homogeneous Transformation  OutputEulerSequence=ZYX  ShowTrVecOutputPort=on  SimulateUsing=Interpreted execution
      settings: SourceProductBaseCode=NV,RO,RR,UV
  Coordinate Transformation Conversion1 : robotcorelib/Coordinate Transformation Conversion  InputRepresentation=Rotation Matrix  InputEulerSequence=ZYX  ShowTrVecInputPort=on  OutputRepresentation=Homogeneous Transformation  OutputEulerSequence=ZYX  ShowTrVecOutputPort=on  SimulateUsing=Interpreted execution
      settings: SourceProductBaseCode=NV,RO,RR,UV
  Grasping Point t : sm_lib/Frames and Transforms/Rigid Transform  TranslationMethod=Cartesian  TranslationStandardOffset=2.5  TranslationLengthUnit=m  TranslationStandardAxis=+X  TranslationCartesianOffset=[2.5 0 0]  TranslationROffset=0  TranslationROffsetUnits=m  TranslationZOffset=0  TranslationZOffsetUnits=m  TranslationThetaOffset=0  TranslationThetaOffsetUnits=deg  RotationMethod=None  RotationAngleUnits=deg  RotationStandardAxis=+Z  RotationAngle=0.0  RotationArbitraryAxis=[0 0 1]  FollAlignAxisA=+X  BaseAlignAxisA=+Y  FollAlignAxisB=+Y  BaseAlignAxisB=+Z  RotationSequenceAxes=FollowerAxes  RotationSequence=XYX  RotationSequenceAngles=[0 0 0]  RotationSequenceAnglesUnits=deg  RotationMatrix=[1 0 0; 0 1 0; 0 0 1]
  Mechanism Configuration1 : sm_lib/Utilities/Mechanism Configuration  UniformGravity=Constant  GravityVector=[0 0 0]  GravityUnits=m/s^2  LinearizationDelta=0.001  JointModeTransitionNonlinearIterations=2
  Mux : Mux  Inputs=6
  Mux4 : Mux  Inputs=3
  Mux8 : Mux  Inputs=3
  PS-Simulink Converter{1..9,13,16,20..22} (14 alike) : nesl_utility/PS-Simulink Converter  PhysicalDomain=network_engine_domain  SubClassName=ps_output  LeftPortType=input  RightPortType=output  PseudoPeriodic=off  Frequencies=[]  Unit=inherit  AffineConversion=off
      settings: SourceProductBaseCode=PW,SS
  Solver Configuration1 : nesl_utility/Solver Configuration  PhysicalDomain=network_engine_domain  SubClassName=solver  LeftPortType=input  RightPortType=generic  Tones=[]  Harmonics=[]  SimulateNoise=off  Profile=off  UseLocalSampling=off  EnableSwitchedLinearOptims=on  FrequencyDomain=off  UseCCode=off  RelTol=0.001  AbsTol=1e-06  MinStep=1e-09  ToWorkspace=off  RevertToSquareIcSolve=off  NumHomotopyIterations=100  PhasorMode=off  PhasorModeNumHarmonics=1  DoDC=off  ResidualTolerance=1e-09  UseLocalSolver=off  LocalSolverChoice=NE_BACKWARD_EULER_ADVANCER  LocalSolverSampleTime=0.001  DoFixedCost=off  MaxNonlinIter=3  MaxModeIter=2  ComputeImpulses=off  ImpulseIterations=2  LinearAlgebra=Sparse  EquationFormulation=NE_TIME_EF  DelaysMemoryBudget=1024  AutomaticFiltering=on  FilteringTimeConstant=0.001  PartitionStorageMethod=AS_NEEDED  PartitionMemoryBudget=1024  PartitionMethod=FAST
      settings: SourceProductBaseCode=PW,SS
  Target : sm_lib/Body Elements/Brick Solid  GraphicAmbientColor=[0.15 0.15 0.15 1.0]  BasedOnType=Mass  BrickDimensions=[0.5, 0.5, 0.5]  BrickDimensionUnits=m  CenterOfMass=[0 0 0]  CenterOfMassUnits=m  GraphicDiffuseColor=[0.5 0.5 0.5]  Density=1000  DensityUnits=kg/m^3  DoExposeReferenceFrame=on  GraphicEmissiveColor=[0.0 0.0 0.0 1.0]  ExportEntireGeometry=on  SerializedFrames=<Frames><Frame><Id>Frame1</Id><Value><Name>F1</Name><Origin><Source>GeometricFeature</Source><FeatureName>+y +z curve</FeatureName></Origin><PrimaryAxis><DefinedDirection>+Z</DefinedDirection><Source>ReferenceFrame</Source><SourceDirection>+Z</SourceDirection><FeatureName></FeatureName></PrimaryAxis><SecondaryAxis><DefinedDirection>+X</DefinedDirection><Source>ReferenceFrame</Source><SourceDirection>+X</SourceDirection><FeatureName></FeatureName></SecondaryAxis></Value></Frame></Frames>  MarkerShape=Sphere  MarkerSize=10  GraphicType=FromGeometry  InertiaType=CalculateFromGeometry  Mass=50  MassUnits=kg  MomentsOfInertia=[1 1 1]  MomentsOfInertiaUnits=kg*m^2  GraphicOpacity=1.0  ProductsOfInertia=[0 0 0]  ProductsOfInertiaUnits=kg*m^2  GraphicShininess=75  GraphicSpecularColor=[0.5 0.5 0.5 1.0]  GraphicVisPropType=SimpleVisualProperties
  Terminator : Terminator
  World Frame1 : sm_lib/Frames and Transforms/World Frame
  g_I_target : Outport
  V_It : Outport  Port=2
  wires:
  Mux8/1 -> Coordinate Transformation Conversion1/2
  PS-Simulink Converter7/1 -> Mux8/1
  PS-Simulink Converter13/1 -> Mux8/3
  PS-Simulink Converter6/1 -> Coordinate Transformation Conversion1/1
  PS-Simulink Converter20/1 -> Mux4/3
  PS-Simulink Converter16/1 -> Mux4/2
  PS-Simulink Converter8/1 -> Mux8/2
  PS-Simulink Converter22/1 -> Mux4/1
  Mux4/1 -> Coordinate Transformation Conversion/2
  PS-Simulink Converter21/1 -> Coordinate Transformation Conversion/1
  Coordinate Transformation Conversion/1 -> g_I_target/1
  Coordinate Transformation Conversion1/1 -> Terminator/1
  PS-Simulink Converter1/1 -> Mux/2
  PS-Simulink Converter2/1 -> Mux/1
  PS-Simulink Converter3/1 -> Mux/3
  PS-Simulink Converter4/1 -> Mux/4
  PS-Simulink Converter5/1 -> Mux/5
  PS-Simulink Converter9/1 -> Mux/6
  Mux/1 -> V_It/1
  connections:
  6-DOF Joint1/LConn1 -- Mechanism Configuration1/RConn1 -- Base Sensing1/LConn1 -- Solver Configuration1/RConn1 -- World Frame1/RConn1
  Base Sensing1/RConn1 -- Target/RConn1 -- 6-DOF Joint1/RConn1
  Base Sensing2/RConn3 -- PS-Simulink Converter7/LConn1
  PS-Simulink Converter21/LConn1 -- Base Sensing1/RConn2
  Grasping Point t/LConn1 -- Base Sensing2/LConn1 -- Target/LConn1
  Base Sensing2/RConn4 -- PS-Simulink Converter8/LConn1
  PS-Simulink Converter22/LConn1 -- Base Sensing1/RConn3
  PS-Simulink Converter20/LConn1 -- Base Sensing1/RConn5
  PS-Simulink Converter16/LConn1 -- Base Sensing1/RConn4
  PS-Simulink Converter6/LConn1 -- Base Sensing2/RConn2
  Grasping Point t/RConn1 -- Base Sensing2/RConn1
  Base Sensing2/RConn5 -- PS-Simulink Converter13/LConn1
  6-DOF Joint1/RConn2 -- PS-Simulink Converter2/LConn1
  6-DOF Joint1/RConn7 -- PS-Simulink Converter9/LConn1
  6-DOF Joint1/RConn6 -- PS-Simulink Converter5/LConn1
  6-DOF Joint1/RConn5 -- PS-Simulink Converter4/LConn1
  6-DOF Joint1/RConn4 -- PS-Simulink Converter3/LConn1
  6-DOF Joint1/RConn3 -- PS-Simulink Converter1/LConn1

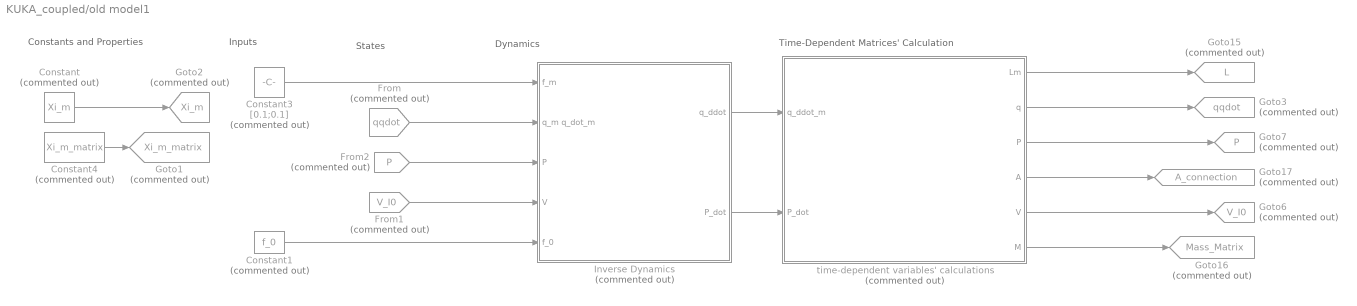
== system KUKA_coupled/old model1 ==
  note: States
  note: Inputs
  note: Time-Dependent Matrices' Calculation
  note: Constants and Properties
  note: Dynamics
  Constant : Constant  Commented=on  Value=Xi_m  VectorParams1D=off
  Constant1 : Constant  Commented=on  Value=f_0  VectorParams1D=off
  Constant3 : Constant  Commented=on  Value=[0.1;0.1]  VectorParams1D=off
  Constant4 : Constant  Commented=on  Value=Xi_m_matrix  VectorParams1D=off
  From : From  Commented=on  GotoTag=qqdot  TagVisibility=global
  From1 : From  Commented=on  GotoTag=V_I0  TagVisibility=global
  From2 : From  Commented=on  GotoTag=P  TagVisibility=global
  Goto1 : Goto  Commented=on  GotoTag=Xi_m_matrix  TagVisibility=global
  Goto15 : Goto  Commented=on  GotoTag=L  TagVisibility=global
  Goto16 : Goto  Commented=on  GotoTag=Mass_Matrix  TagVisibility=global
  Goto17 : Goto  Commented=on  GotoTag=A_connection  TagVisibility=global
  Goto2 : Goto  Commented=on  GotoTag=Xi_m  TagVisibility=global
  Goto3 : Goto  Commented=on  GotoTag=qqdot  TagVisibility=global
  Goto6 : Goto  Commented=on  GotoTag=V_I0  TagVisibility=global
  Goto7 : Goto  Commented=on  GotoTag=P  TagVisibility=global
  Inverse Dynamics : Subsystem  Commented=on
  time-dependent variables' calculations : Subsystem  Commented=on
  wires:
  Constant3/1 -> Inverse Dynamics/1(f_m)
  From1/1 -> Inverse Dynamics/4(V)
  time-dependent variables' calculations/6(M) -> Goto16/1
  Inverse Dynamics/2(P_dot) -> time-dependent variables' calculations/2(P_dot)
  time-dependent variables' calculations/2(q) -> Goto3/1
  Constant1/1 -> Inverse Dynamics/5(f_0)
  Constant/1 -> Goto2/1
  time-dependent variables' calculations/1(Lm) -> Goto15/1
  time-dependent variables' calculations/3(P) -> Goto7/1
  From/1 -> Inverse Dynamics/2(q_m q_dot_m)
  Constant4/1 -> Goto1/1
  time-dependent variables' calculations/5(V) -> Goto6/1
  Inverse Dynamics/1(q_ddot) -> time-dependent variables' calculations/1(q_ddot_m)
  time-dependent variables' calculations/4(A) -> Goto17/1
  From2/1 -> Inverse Dynamics/3(P)

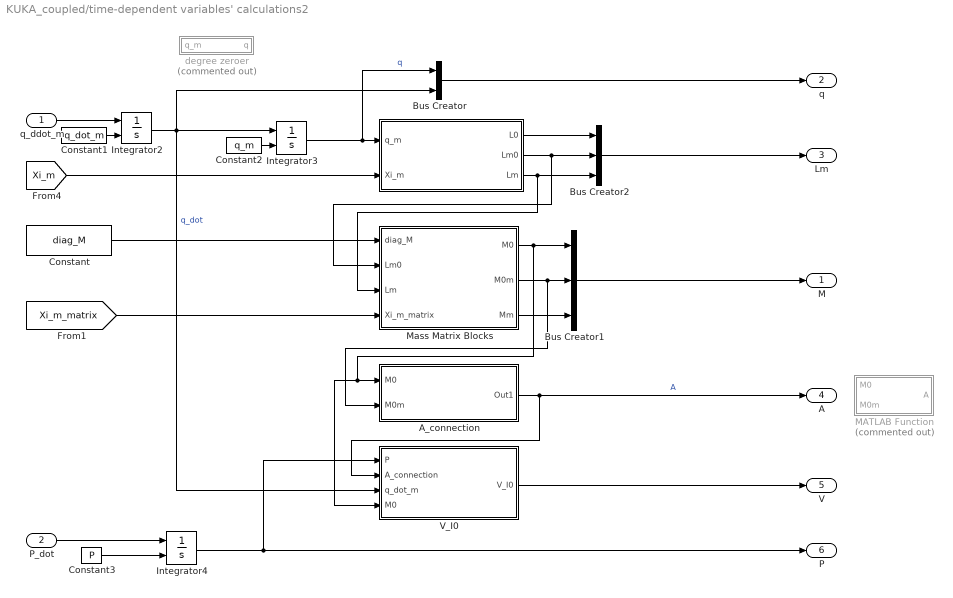
== system KUKA_coupled/time-dependent variables' calculations2 ==
  q_ddot_m : Inport
  P_dot : Inport  Port=2
  " " : MATLAB Function  TreatAsAtomicUnit=on
  A_connection : Subsystem
  Bus Creator : BusCreator  Inputs=2
  Bus Creator1 : BusCreator  Inputs=3
  Bus Creator2 : BusCreator  Inputs=3
  Constant : Constant  Value=diag_M  VectorParams1D=off
  Constant1 : Constant  Value=q_dot_m  VectorParams1D=off
  Constant2 : Constant  Value=q_m  VectorParams1D=off
  Constant3 : Constant  Value=P  VectorParams1D=off
  Integrator2 : Integrator  InitialConditionSource=external  InitialCondition=q_dot_m
  Integrator3 : Integrator  InitialConditionSource=external
  Integrator4 : Integrator  InitialConditionSource=external
  MATLAB Function : MATLAB Function  Commented=on  TreatAsAtomicUnit=on
  Mass Matrix Blocks : Subsystem
  V_I0 : MATLAB Function  TreatAsAtomicUnit=on
  degree zeroer : MATLAB Function  Commented=on  TreatAsAtomicUnit=on
  M : Outport
  q : Outport  Port=2
  Lm : Outport  Port=3
  A : Outport  Port=4
  V : Outport  Port=5
  P : Outport  Port=6
  wires:
  Mass Matrix Blocks/3(Mm) -> Bus Creator1/3
  Integrator2/1 -> V_I0/3(q_dot_m), Bus Creator/2, Integrator3/1  "q_dot"
  q_ddot_m/1 -> Integrator2/1
  " "/1(L0) -> Bus Creator2/1
  " "/3(Lm) -> Mass Matrix Blocks/3(Lm), Bus Creator2/3
  " "/2(Lm0) -> Mass Matrix Blocks/2(Lm0), Bus Creator2/2
  Constant/1 -> Mass Matrix Blocks/1(diag_M)
  [Xi_m_matrix] -> Mass Matrix Blocks/4(Xi_m_matrix)
  [Xi_m] -> " "/2(Xi_m)
  Integrator3/1 -> Bus Creator/1, " "/1(q_m)  "q"
  Bus Creator/1 -> q/1
  Constant1/1 -> Integrator2/2
  Constant2/1 -> Integrator3/2
  Bus Creator2/1 -> Lm/1
  Bus Creator1/1 -> M/1
  Mass Matrix Blocks/2(M0m) -> A_connection/2(M0m), Bus Creator1/2
  Mass Matrix Blocks/1(M0) -> V_I0/4(M0), A_connection/1(M0), Bus Creator1/1
  A_connection/1(Out1) -> V_I0/2(A_connection), A/1  "A"
  V_I0/1(V_I0) -> V/1
  P_dot/1 -> Integrator4/1
  Integrator4/1 -> V_I0/1(P), P/1
  Constant3/1 -> Integrator4/2

== system KUKA_coupled/Inverse Dynamics2/Euler Poincare ==
  P : Inport
  V : Inport  Port=2
  f_0 : Inport  Port=3
  Add : Sum  Inputs=-+
  Constant : Constant  Value=iota0
  Constant1 : Constant  Commented=on  Value=eye(6,6)
  MATLAB Function : MATLAB Function  TreatAsAtomicUnit=on
  Matrix Multiply : Product  Multiplication=Matrix(*)
  To Workspace : ToWorkspace  VariableName=simout  SaveFormat=Timeseries  SampleTime=-1
  Transpose : Math  Operator=transpose  SaturateOnIntegerOverflow=on
  adj_low_P : MATLAB Function  Commented=on  TreatAsAtomicUnit=on
  P_dot : Outport
  wires:
  P/1 -> Matrix Multiply/2
  MATLAB Function/1(adj_low) -> Transpose/1
  V/1 -> MATLAB Function/1(V)
  Transpose/1 -> To Workspace/1, Matrix Multiply/1
  Matrix Multiply/1 -> Add/1
  f_0/1 -> Add/2
  Add/1 -> P_dot/1
  Constant/1 -> MATLAB Function/2(iota0)

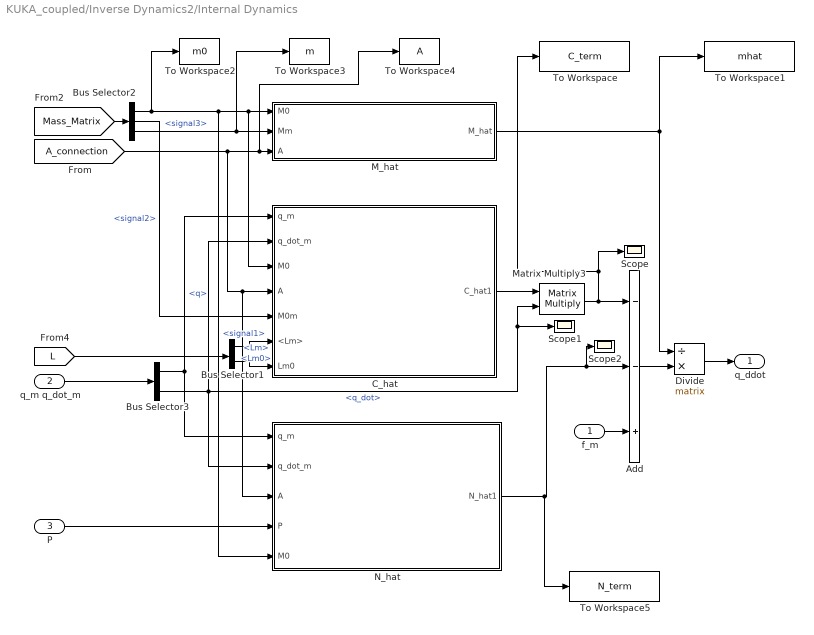
== system KUKA_coupled/Inverse Dynamics2/Internal Dynamics ==
  f_m : Inport
  q_m q_dot_m : Inport  Port=2
  P : Inport  Port=3
  Add : Sum  Inputs=--+
  Bus Selector1 : BusSelector  OutputSignals=Lm,Lm0
  Bus Selector2 : BusSelector  OutputSignals=signal1,signal2,signal3
  Bus Selector3 : BusSelector  OutputSignals=q,q_dot
  C_hat : Subsystem
  Divide : Product  Inputs=/*  Multiplication=Matrix(*)
  M_hat : MATLAB Function  TreatAsAtomicUnit=on
  Matrix Multiply3 : Product  Multiplication=Matrix(*)
  N_hat : Subsystem
  Scope : Scope
  Scope1 : Scope
  Scope2 : Scope
  To Workspace : ToWorkspace  VariableName=C_term  SaveFormat=Timeseries  SampleTime=-1
  To Workspace1 : ToWorkspace  VariableName=mhat  SaveFormat=Timeseries  SampleTime=-1
  To Workspace2 : ToWorkspace  VariableName=m0  SaveFormat=Timeseries  SampleTime=-1
  To Workspace3 : ToWorkspace  VariableName=m  SaveFormat=Timeseries  SampleTime=-1
  To Workspace4 : ToWorkspace  VariableName=A  SaveFormat=Timeseries  SampleTime=-1
  To Workspace5 : ToWorkspace  VariableName=N_term  SaveFormat=Timeseries  SampleTime=-1
  q_ddot : Outport
  wires:
  Bus Selector3/1 -> C_hat/1(q_m), N_hat/1(q_m)  "<q>"
  f_m/1 -> Add/3
  Bus Selector2/3 -> To Workspace3/1, M_hat/2(Mm)  "<signal3>"
  q_m q_dot_m/1 -> Bus Selector3/1
  C_hat/1(C_hat1) -> Matrix Multiply3/1
  [A_connection] -> To Workspace4/1, M_hat/3(A), C_hat/4(A), N_hat/3(A)
  [L] -> Bus Selector1/1
  Bus Selector2/1 -> N_hat/5(M0), M_hat/1(M0), C_hat/3(M0), To Workspace2/1  "<signal1>"
  [Mass_Matrix] -> Bus Selector2/1
  Bus Selector3/2 -> N_hat/2(q_dot_m), C_hat/2(q_dot_m), Matrix Multiply3/2, Scope1/1  "<q_dot>"
  Divide/1 -> q_ddot/1
  Bus Selector2/2 -> C_hat/5(M0m)  "<signal2>"
  Bus Selector1/2 -> C_hat/7(Lm0)  "<Lm0>"
  Bus Selector1/1 -> C_hat/6(<Lm>)  "<Lm>"
  Matrix Multiply3/1 -> To Workspace/1, Scope/1, Add/1
  Add/1 -> Divide/2
  M_hat/1(M_hat) -> To Workspace1/1, Divide/1
  P/1 -> N_hat/4(P)
  N_hat/1(N_hat1) -> To Workspace5/1, Scope2/1, Add/2

== system KUKA_coupled/Space Manipulator1/fixed base ==
  iiwa_link_0 : Subsystem
  world_iiwa_joint : sm_lib/Joints/Weld Joint  JointMode=Normal  SenseConstraintForce=off  SenseConstraintForceX=off  SenseConstraintForceY=off  SenseConstraintForceZ=off  SenseConstraintTorque=off  SenseConstraintTorqueX=off  SenseConstraintTorqueY=off  SenseConstraintTorqueZ=off  SenseTotalForce=off  SenseTotalForceX=off  SenseTotalForceY=off  SenseTotalForceZ=off  SenseTotalTorque=off  SenseTotalTorqueX=off  SenseTotalTorqueY=off  SenseTotalTorqueZ=off  CompositeWrenchDir=FollowerOnBase  CompositeWrenchFrame=BaseFrame
  F1 : PMIOPort  Side=Right
  Conn2 : PMIOPort  Port=2  Side=Left
  connections:
  iiwa_link_0/LConn1 -- world_iiwa_joint/RConn1
  Conn2/RConn1 -- world_iiwa_joint/LConn1
  F1/RConn1 -- iiwa_link_0/RConn1

== system KUKA_coupled/Space Manipulator1/iiwa_link_ee ==
  ReferenceFrame : sm_lib/Frames and Transforms/Reference Frame
  F : PMIOPort  Side=Left
  connections:
  ReferenceFrame/RConn1 -- F/RConn1

== system KUKA_coupled/Space Manipulator1/iiwa_link_ee_kuka ==
  ReferenceFrame : sm_lib/Frames and Transforms/Reference Frame
  F : PMIOPort  Side=Left
  connections:
  ReferenceFrame/RConn1 -- F/RConn1

== system KUKA_coupled/Space Manipulator1/join//link 1 ==
  iiwa_joint_1 : sm_lib/Joints/Revolute Joint  JointMode=Normal  SenseConstraintForce=off  SenseConstraintForceX=off  SenseConstraintForceY=off  SenseConstraintForceZ=off  SenseConstraintTorque=off  SenseConstraintTorqueX=off  SenseConstraintTorqueY=off  SenseConstraintTorqueZ=off  SenseTotalForce=off  SenseTotalForceX=off  SenseTotalForceY=off  SenseTotalForceZ=off  SenseTotalTorque=off  SenseTotalTorqueX=off  SenseTotalTorqueY=off  SenseTotalTorqueZ=off  CompositeWrenchDir=FollowerOnBase  CompositeWrenchFrame=BaseFrame  EquilibriumPosition=0  EquilibriumPositionUnits=deg  SpringStiffness=0  SpringStiffnessUnits=N*m/deg  DampingCoefficient=0.5  DampingCoefficientUnits=kg*m^2/(rad*s)  TorqueActuationMode=InputTorque  MotionActuationMode=ComputedMotion  SensePosition=on  SenseVelocity=on  SenseAcceleration=on  SenseTorqueForce=off  SenseLowerLimitTorqueForce=off  SenseUpperLimitTorqueForce=off  LowerLimitSpecify=on  LowerLimitBound=-2.96705972839  LowerLimitBoundUnits=rad  LowerLimitStiffness=1e4  LowerLimitStiffnessUnits=N*m/deg  LowerLimitDamping=10  LowerLimitDampingUnits=N*m/(deg/s)  LowerLimitTransitionRegionWidth=0.1  LowerLimitTransitionRegionWidthUnits=deg  UpperLimitSpecify=on  UpperLimitBound=2.96705972839  UpperLimitBoundUnits=rad  UpperLimitStiffness=1e4  UpperLimitStiffnessUnits=N*m/deg  UpperLimitDamping=10  UpperLimitDampingUnits=N*m/(deg/s)  UpperLimitTransitionRegionWidth=0.1  UpperLimitTransitionRegionWidthUnits=deg  PositionTargetSpecify=on  PositionTargetPriority=High  PositionTargetValue=0  PositionTargetValueUnits=deg  VelocityTargetSpecify=off  VelocityTargetPriority=High  VelocityTargetValue=0  VelocityTargetValueUnits=deg/s
  iiwa_link_1 : Subsystem
  f1 : PMIOPort  Side=Left
  b : PMIOPort  Port=2  Side=Left
  F1 : PMIOPort  Port=3  Side=Right
  q1 : PMIOPort  Port=4  Side=Right
  qd1 : PMIOPort  Port=5  Side=Right
  qdd1 : PMIOPort  Port=6  Side=Right
  connections:
  iiwa_joint_1/RConn1 -- iiwa_link_1/LConn1
  iiwa_joint_1/LConn1 -- b/RConn1
  iiwa_joint_1/RConn2 -- q1/RConn1
  f1/RConn1 -- iiwa_joint_1/LConn2
  iiwa_joint_1/RConn3 -- qd1/RConn1
  iiwa_joint_1/RConn4 -- qdd1/RConn1
  F1/RConn1 -- iiwa_link_1/RConn1
